simulink model "Grid_ModelSimVSGConB"  (R2025b)
settings: Solver=daessc  StartTime=0.0  StopTime=10  MaxStep=1e-5  RelTol=1e-3
InitFcn:
  | Grid_ModelSimV1
values from neighbouring files (symbols this model uses):
  a = 0.5    [Grid_ModelSimV1.m]
  b = (beta*gamma)/(beta + gamma - a)    [Grid_ModelSimV1.m]
  c = (beta + gamma - a)/mp    [Grid_ModelSimV1.m]
  D1 = Moh_Dp/Moh_Sbase    (= 0.2546)    [Grid_ModelSimV1.m]
  D2 = 0.4    [Grid_ModelSimV1.m]
  delta1_0 = delta1PCC0 + atan2(      P12_0*X1/V1PCCmag0,      V1PCCmag0 + Q12_0*X1/V1PCCmag0 )    [Grid_ModelSimV1.m]
  delta2_0 = delta2PCC0 + atan2(      Pm2_0*X2/V2PCCmag0,      V2PCCmag0 + Q21_0*X2/V2PCCmag0 )    [Grid_ModelSimV1.m]
  Dw1_0 = 0    [Grid_ModelSimV1.m]
  Dw2_0 = 0    [Grid_ModelSimV1.m]
  E2_0 = hypot(      Pm2_0*X2/V2PCCmag0,      V2PCCmag0 + Q21_0*X2/V2PCCmag0 )    [Grid_ModelSimV1.m]
  H1 = J*omega_nom^2/2    (= 39.9916370332)    [Grid_ModelSimV1.m]
  H2 = 12    [Grid_ModelSimV1.m]
  Imax = 1.20    (= 1.2)    [Grid_ModelSimV1.m]
  J = Moh_J/Moh_Sbase    (= 0.0008104)    [Grid_ModelSimV1.m]
  Ki = 0.5    [Grid_ModelSimV1.m]
  Kiq = Moh_Kiq*Moh_Sbase/Moh_Vbase    [Grid_ModelSimV1.m]
  Lf = 1e-3    (= 0.001)    [Grid_ModelSimV1.m]
  LimitEnable = 1    [Grid_ModelSimV1.m]
  Ls = Xs/ws    [Grid_ModelSimV1.m]
  Ls_line = Xs_line/ws    [Grid_ModelSimV1.m]
  nq = Moh_nq*Moh_Sbase/Moh_Vbase    [Grid_ModelSimV1.m]
  omega_nom = ws    (= 314.159265359)    [Grid_ModelSimV1.m]
  Pload_0 = P12_0    (= 1)    [Grid_ModelSimV1.m]
  Qref = 0.0    (= 0)    [Grid_ModelSimV1.m]
  Rf = 1.0    (= 1)    [Grid_ModelSimV1.m]
  RLFault = 0    [Grid_ModelSimV1.m]
  Rs = Zs_mag/sqrt(1 + XR_grid^2)    [Grid_ModelSimV1.m]
  Rs_line = GridLineFraction*Rs    [Grid_ModelSimV1.m]
  SolidFault = 0    [Grid_ModelSimV1.m]
  ws = 2*pi*f    (= 314.159265359)    [Grid_ModelSimV1.m]
  X1 = Xtf_src_total_pu    (= 0.15)    [Grid_ModelSimV1.m]
libraries: nesl_utility x87, ee_lib x78, fl_lib x40, eePowerMeasurement x7
(part 6 of 6)

== matlab function Grid_ModelSimVSGConB/Controller B with Limiter/MATLAB Function2 ==
  data: Ecmd input; Eactual output; deltaActual output; deltaCmd input; Vpcc input; deltaPCC input; kApplied input; LimitEnable input; LimiterActive output; scale output; deltaPCC_used output

function [Eactual,deltaActual,LimiterActive,scale,deltaPCC_used] = ...
    CurrentLimiter(Ecmd,deltaCmd,Vpcc,deltaPCC,kApplied,LimitEnable)

% ============================================================
% PHASOR CURRENT LIMITER
%
% Scaling is controlled externally by CurrentScaleController.
%
% Inputs:
% Ecmd        - commanded voltage magnitude [pu]
% deltaCmd    - commanded source angle [rad]
% Vpcc        - measured PCC voltage magnitude [pu]
% deltaPCC    - measured PCC phase angle [rad]
% kApplied    - scaling from external discrete controller
% LimitEnable - limiter enable (0 or 1)
%
% Outputs:
% Eactual       - applied source voltage magnitude [pu]
% deltaActual   - applied source voltage angle [rad]
% LimiterActive - limiter status
% scale         - applied scaling factor
% deltaPCC_used - corrected PCC angle used by limiter
% ============================================================

%% PCC angle settings

thetaOffset   = 0;
deltaThetaRef = 0.15;

Vlow  = 0.20;
Vhigh = 0.80;

%% External current-limiting scale

if LimitEnable > 0.5

    % Use scale generated by CurrentScaleController
    scale = min(1,max(0,kApplied));

else

    % Limiter disabled: full pass-through
    scale = 1;

end

LimiterActive = (LimitEnable > 0.5) && (scale < 0.999);

%% Correct PCC angle reference

deltaPCC_meas = deltaPCC - thetaOffset;

relMeasured = atan2( ...
    sin(deltaPCC_meas - deltaCmd), ...
    cos(deltaPCC_meas - deltaCmd));

%% Low-voltage angle fallback

relFallback = -deltaThetaRef;

%% Smooth low-voltage angle blending

% Voltage-based phase reliability
alphaV = (Vpcc - Vlow)/(Vhigh - Vlow);
alphaV = min(1,max(0,alphaV));

% Suppress PCC phase feedback during strong limiting
alphaK = (scale - 0.80)/0.20;
alphaK = min(1,max(0,alphaK));

% Combined blending factor
alpha = alphaV;

relError = atan2( ...
    sin(relMeasured - relFallback), ...
    cos(relMeasured - relFallback));

relUsed = relFallback + alpha*relError;

deltaPCC_used = deltaCmd + relUsed;

%% Build PCC voltage phasor in local reference

Vpcc_local = Vpcc*exp(1j*relUsed);

%% Apply external scaling to voltage phasor

Eactual_local = ...
    Vpcc_local + scale*(Ecmd - Vpcc_local);

%% Calculate magnitude and phase

Eactual = abs(Eactual_local);

deltaCorrection = angle(Eactual_local);

deltaActual = deltaCmd + deltaCorrection;

%% Exact bypass when limiter is inactive

if scale >= 1

    Eactual = Ecmd;
    deltaActual = deltaCmd;

end

end

== matlab function Grid_ModelSimVSGConB/Controller B with Limiter/MATLAB Function3 ==
  data: u input; y output
function y = fcn(u)

y = 1 - u;

== matlab function Grid_ModelSimVSGConB/Controller C with Limiter/MATLAB Function1 ==
  data: Imeas input; kNext output; Imax input; LimitEnable input; kPrev input

function kNext = CurrentScaleController(Imeas,Imax,LimitEnable,kPrev)

% Discrete exponential current limiter
% All currents in pu

Ts = 1e-4;          % Sample time [s]

Kdown = 10;         % Current reduction gain
Kup   = 4;          % Recovery gain

Kmin = 0.02;        % Minimum voltage scaling
releaseMargin = 0.05;

Ion  = Imax;
Ioff = max(Imax-releaseMargin,0);

% Disable limiter
if LimitEnable < 0.5
    kNext = 1;
    return;
end

% CURRENT ABOVE LIMIT - exponentially reduce scaling
if Imeas > Ion

    excess = Imeas-Ion;

    kNext = kPrev*exp(-Kdown*excess*Ts);

% CURRENT BELOW RELEASE THRESHOLD - recover gradually
elseif Imeas < Ioff

    kNext = 1-(1-kPrev)*exp(-Kup*Ts);

% CURRENT WITHIN DEADBAND - hold previous scaling
else

    kNext = kPrev;

end

% Bound scaling
kNext = min(1,max(Kmin,kNext));

end

== matlab function Grid_ModelSimVSGConB/Controller C with Limiter/MATLAB Function2 ==
  data: Ecmd input; Eactual output; deltaActual output; deltaCmd input; Vpcc input; deltaPCC input; kApplied input; LimitEnable input; LimiterActive output; scale output; deltaPCC_used output

function [Eactual,deltaActual,LimiterActive,scale,deltaPCC_used] = ...
    CurrentLimiter(Ecmd,deltaCmd,Vpcc,deltaPCC,kApplied,LimitEnable)

% ============================================================
% PHASOR CURRENT LIMITER
%
% Scaling is controlled externally by CurrentScaleController.
%
% Inputs:
% Ecmd        - commanded voltage magnitude [pu]
% deltaCmd    - commanded source angle [rad]
% Vpcc        - measured PCC voltage magnitude [pu]
% deltaPCC    - measured PCC phase angle [rad]
% kApplied    - scaling from external discrete controller
% LimitEnable - limiter enable (0 or 1)
%
% Outputs:
% Eactual       - applied source voltage magnitude [pu]
% deltaActual   - applied source voltage angle [rad]
% LimiterActive - limiter status
% scale         - applied scaling factor
% deltaPCC_used - corrected PCC angle used by limiter
% ============================================================

%% PCC angle settings

thetaOffset   = 0;
deltaThetaRef = 0.15;

Vlow  = 0.20;
Vhigh = 0.80;

%% External current-limiting scale

if LimitEnable > 0.5

    % Use scale generated by CurrentScaleController
    scale = min(1,max(0,kApplied));

else

    % Limiter disabled: full pass-through
    scale = 1;

end

LimiterActive = (LimitEnable > 0.5) && (scale < 0.999);

%% Correct PCC angle reference

deltaPCC_meas = deltaPCC - thetaOffset;

relMeasured = atan2( ...
    sin(deltaPCC_meas - deltaCmd), ...
    cos(deltaPCC_meas - deltaCmd));

%% Low-voltage angle fallback

relFallback = -deltaThetaRef;

%% Smooth low-voltage angle blending

% Voltage-based phase reliability
alphaV = (Vpcc - Vlow)/(Vhigh - Vlow);
alphaV = min(1,max(0,alphaV));

% Suppress PCC phase feedback during strong limiting
alphaK = (scale - 0.80)/0.20;
alphaK = min(1,max(0,alphaK));

% Combined blending factor
alpha = alphaV;

relError = atan2( ...
    sin(relMeasured - relFallback), ...
    cos(relMeasured - relFallback));

relUsed = relFallback + alpha*relError;

deltaPCC_used = deltaCmd + relUsed;

%% Build PCC voltage phasor in local reference

Vpcc_local = Vpcc*exp(1j*relUsed);

%% Apply external scaling to voltage phasor

Eactual_local = ...
    Vpcc_local + scale*(Ecmd - Vpcc_local);

%% Calculate magnitude and phase

Eactual = abs(Eactual_local);

deltaCorrection = angle(Eactual_local);

deltaActual = deltaCmd + deltaCorrection;

%% Exact bypass when limiter is inactive

if scale >= 1

    Eactual = Ecmd;
    deltaActual = deltaCmd;

end

end
